simulink model "Controlador"  (R2026b)
settings: Solver=VariableStepAuto
values from neighbouring files (symbols this model uses):
  theta_init = pi - 20 * pi/180    (= 2.79252680319)    [Pendulo_Invertido.m]
  x_init = -0.35    [Pendulo_Invertido.m]
libraries: eeGeneralControl x1, mcbhdlpositiondecoderlib x1
settings Model: Creator=fedeb  LastModifiedBy=fedeb

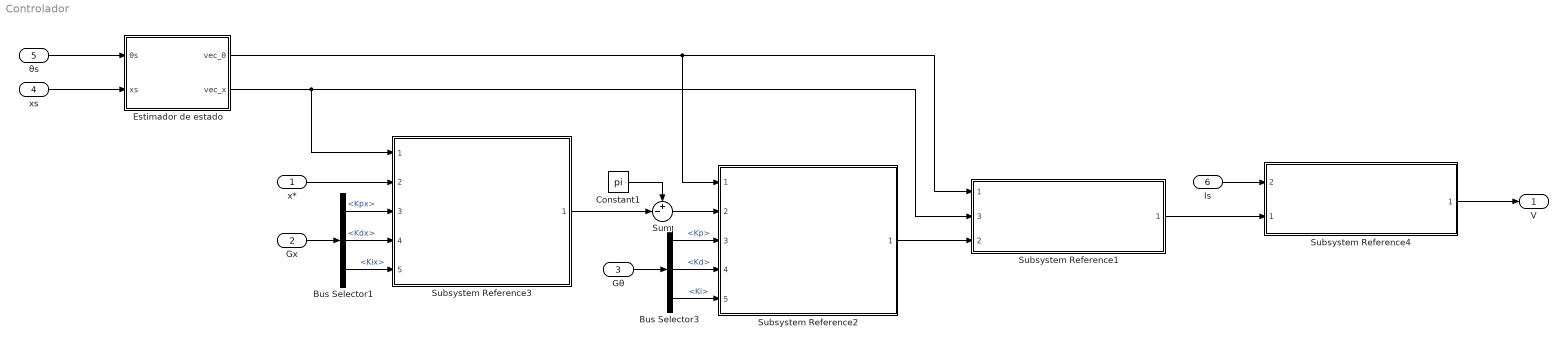
== system Controlador ==
  x* : Inport
  Gx : Inport  Port=2
  Gθ : Inport  Port=3
  xs : Inport  Port=4
  θs : Inport  Port=5
  Ⅰs : Inport  Port=6
  Bus Selector1 : BusSelector  OutputSignals=Kpx,Kdx,Kix
  Bus Selector3 : BusSelector  OutputSignals=Kp,Kd,Ki
  Constant1 : Constant  Value=pi
  Estimador de estado : Subsystem
  Subsystem Reference1 : Subsystem  ReferencedSubsystem=RetroalimentacionNoLineal_v2
      settings: PortSchema="{\"entries\":[{\"content\":{\"sides\":[{\"content\":{\"connectorIds\":[\"In1\",\"In3\",\"In2\"]},\"type\":\"ConnectorPlacement.EquallySpacedRectSide\",\"uuid\":\"610c099f-3880-471b-9338-edcc5bdfe28a\"},{\"content\":{\"connectorIds\":[\"Out1\"],\"side\":\"RIGHT\"},\"type\":\"ConnectorPlacement.EquallySpacedRectSide\",\"uuid\":\"8e1fd953-d966-4147-a248-c67292fa34b0\"},{\"content\":{\"side\":\"TOP\"},\"type\":\"ConnectorPlacement.EquallySpacedRectSide\",\"uuid\":\"9b639fd1-3713-4a39-9913-6689bdfa49a0\"}]},\"type\":\"ConnectorPlacement.EquallySpacedConnector\",\"uuid\":\"38458ebd-b19e-423d-b29f-e53f185d6ba5\"}],\"packageUris\":[\"http://schema.mathworks.com/mf0/Connector/R2020b\"],\"version\":\"1.0\"}"
  Subsystem Reference2 : Subsystem  ReferencedSubsystem=ControladorAngularPID
  Subsystem Reference3 : Subsystem  ReferencedSubsystem=ControladorTraslacionPID
  Subsystem Reference4 : Subsystem  ReferencedSubsystem=ControladorCorriente
      settings: PortSchema="{\"entries\":[{\"content\":{\"sides\":[{\"content\":{\"connectorIds\":[\"In2\",\"In1\"]},\"type\":\"ConnectorPlacement.EquallySpacedRectSide\",\"uuid\":\"7c00aa9d-1e51-4f60-8af2-27b9c8516297\"},{\"content\":{\"connectorIds\":[\"Out1\"],\"side\":\"RIGHT\"},\"type\":\"ConnectorPlacement.EquallySpacedRectSide\",\"uuid\":\"c8dedb51-8fa1-460c-b8a3-b96998a053c0\"},{\"content\":{\"side\":\"TOP\"},\"type\":\"ConnectorPlacement.EquallySpacedRectSide\",\"uuid\":\"3864dafc-18b8-4237-b97a-b4120ef67b07\"}]},\"type\":\"ConnectorPlacement.EquallySpacedConnector\",\"uuid\":\"76c7a363-6b22-4894-ad00-ddf8ba6f7225\"}],\"packageUris\":[\"http://schema.mathworks.com/mf0/Connector/R2020b\"],\"version\":\"1.0\"}"
  Sum : Sum  Inputs=+-|
  V : Outport
  wires:
  θs/1 -> Estimador de estado/1(θs)
  Estimador de estado/1(vec_θ) -> Subsystem Reference1/1, Subsystem Reference2/1
  xs/1 -> Estimador de estado/2(xs)
  Estimador de estado/2(vec_x) -> Subsystem Reference3/1, Subsystem Reference1/3
  Subsystem Reference3/1 -> Sum/2
  Bus Selector1/3 -> Subsystem Reference3/5  "<Kix>"
  Bus Selector1/1 -> Subsystem Reference3/3  "<Kpx>"
  Bus Selector1/2 -> Subsystem Reference3/4  "<Kdx>"
  Sum/1 -> Subsystem Reference2/2
  x*/1 -> Subsystem Reference3/2
  Bus Selector3/1 -> Subsystem Reference2/3  "<Kp>"
  Bus Selector3/2 -> Subsystem Reference2/4  "<Kd>"
  Gθ/1 -> Bus Selector3/1
  Bus Selector3/3 -> Subsystem Reference2/5  "<Ki>"
  Gx/1 -> Bus Selector1/1
  Constant1/1 -> Sum/1
  Subsystem Reference2/1 -> Subsystem Reference1/2
  Ⅰs/1 -> Subsystem Reference4/2
  Subsystem Reference1/1 -> Subsystem Reference4/1
  Subsystem Reference4/1 -> V/1

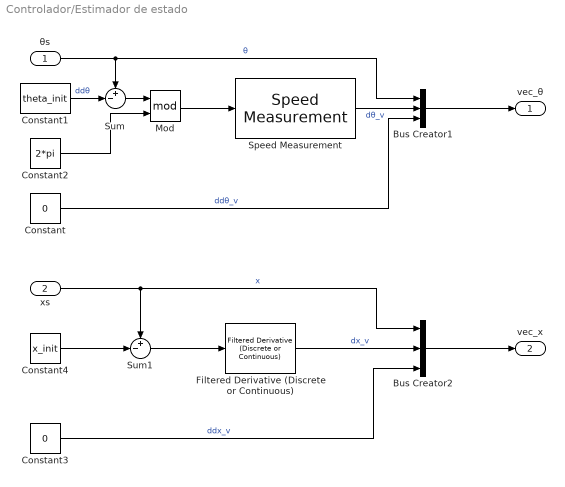
== system Controlador/Estimador de estado ==
  θs : Inport
  xs : Inport  Port=2
  Bus Creator1 : BusCreator  Inputs=3
  Bus Creator2 : BusCreator  Inputs=3
  Constant : Constant  Value=0
  Constant1 : Constant  Value=theta_init
  Constant2 : Constant  Value=2*pi
  Constant3 : Constant  Value=0
  Constant4 : Constant  Value=x_init
  Filtered Derivative (Discrete or Continuous) : eeGeneralControl/Filtered Derivative (Discrete or Continuous)  K=1  T=0.1  B=inf  A=-inf  minRatio=10  init_option=Specify as parameter  x0=dx_init  Ts=-1
      settings: LibrarySourceBlock=|
      | ee_sl_lib/General Control/Filtered Derivative
      | (Discrete or Continuous)
  Mod : Math  Operator=mod
  Speed Measurement : mcbhdlpositiondecoderlib/Speed Measurement  PositionUnit=Radians  PositionScalingDatatype=uint32  SpeedCalculationMode=Maximum application speed  SampleTimeAsync=Ts_medicion  MaximumApplicationSpeed=1000  SpeedResolution=5e-6  DelayLength=29  MaximumMeasurableSpeed=1000  MeasurableSpeedResolution=4.6566e-07  SpeedUnit=Radians/Sec  PerUnitSpeed=1000  SpeedDataType=single
      settings: LibrarySourceBlock=mcbhdllib/Sensor Decoders/Speed Measurement
  Sum : Sum  Inputs=+-|
  Sum1 : Sum  Inputs=+-|
  vec_θ : Outport
  vec_x : Outport  Port=2
  wires:
  Speed Measurement/1 -> Bus Creator1/2  "dθ_v"
  Bus Creator1/1 -> vec_θ/1
  θs/1 -> Bus Creator1/1, Sum/1  "θ"
  Constant/1 -> Bus Creator1/3  "ddθ_v"
  Constant1/1 -> Sum/2  "ddθ"
  Sum/1 -> Mod/1
  Constant2/1 -> Mod/2
  Mod/1 -> Speed Measurement/1
  Constant3/1 -> Bus Creator2/3  "ddx_v"
  Filtered Derivative (Discrete or Continuous)/1 -> Bus Creator2/2  "dx_v"
  Bus Creator2/1 -> vec_x/1
  xs/1 -> Bus Creator2/1, Sum1/1  "x"
  Constant4/1 -> Sum1/2
  Sum1/1 -> Filtered Derivative (Discrete or Continuous)/1
